simulink model "AEC_model"  (R2025b)
settings: Solver=FixedStepDiscrete  StartTime=0.0  StopTime=5  FixedStep=1/8000  RelTol=1e-3
undefined symbols (not defined in the file): hEcho
libraries: dspadpt3 x1
settings Model: Creator=MAITHRI  LastModifiedBy=MAITHRI

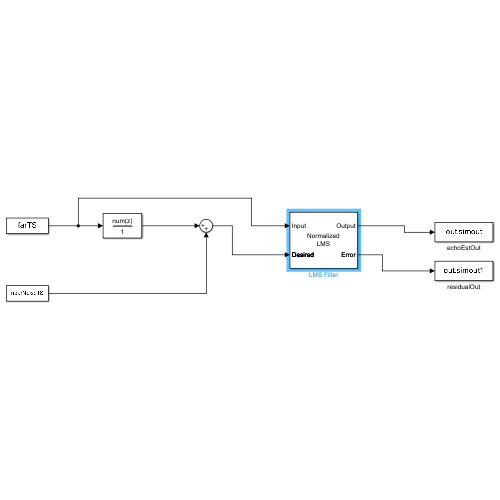
[thumbnail: Simulink's stored preview of the top-level diagram]
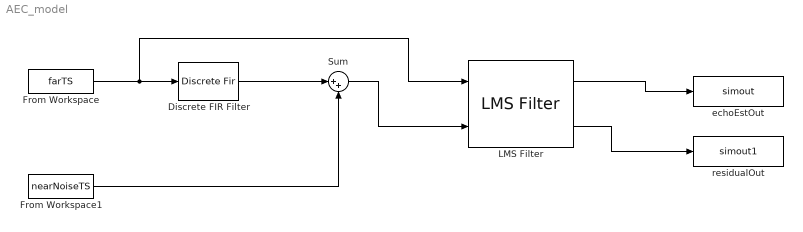
== system AEC_model ==
  Discrete FIR Filter : DiscreteFir  Coefficients=hEcho
  From Workspace : FromWorkspace  VariableName=farTS  SampleTime=1/8000  Interpolate=off  OutputAfterFinalValue=Setting to zero
  From Workspace1 : FromWorkspace  VariableName=nearNoiseTS  SampleTime=1/8000  Interpolate=off  OutputAfterFinalValue=Setting to zero
  LMS Filter : dspadpt3/LMS Filter  Algo=Normalized LMS  L=256  stepflag=Dialog  mu=muStep  leakage=1.0  ic=0  Adapt=off  resetflag=None  weights=off  addnparflag=off  roundingMode=Floor  overflowMode=off
      settings: LibrarySourceBlock=AdaptiveEchoCancellation/LMS Filter
  Sum : Sum  Inputs=|++
  echoEstOut : ToWorkspace  VariableName=simout  SaveFormat=Timeseries  SampleTime=-1
  residualOut : ToWorkspace  VariableName=simout1  SaveFormat=Timeseries  SampleTime=-1
  wires:
  LMS Filter/1 -> echoEstOut/1
  Sum/1 -> LMS Filter/2
  Discrete FIR Filter/1 -> Sum/1
  From Workspace1/1 -> Sum/2
  From Workspace/1 -> LMS Filter/1, Discrete FIR Filter/1
  LMS Filter/2 -> residualOut/1
